simulink model "Robot_model_P_Control_ZOH_2025b"  (R2026a)
settings: Solver=VariableStepAuto  StopTime=10
values from neighbouring files (symbols this model uses):
  B = D * L    (= 9.682e-08)    [measurements.m]    (also in run_simulink.m = 0.15; run_simulink_PI_Controller.m = 0.15; run_simulink_turnrate_Controller.m = 0.15; run_simulink_turnrate_Controller_Heading.m = 0.15)
  D = 0.0000188    (= 1.88e-05)    [measurements.m]    (also in motor_model_m.m = 5e-05; run_simulink.m = 5e-05; run_simulink_PI_Controller.m = 5e-05; run_simulink_turnrate_Controller.m = 5e-05)
  J = -b / a    (= 2.25042607204e-06)    [measurements.m]    (also in motor_model_m.m = 5.56231644013e-06; run_simulink.m = 5.56231644013e-06; run_simulink_PI_Controller.m = 5.56231644013e-06; run_simulink_turnrate_Controller.m = 5.56231644013e-06)
  Kb = Kt    (= 0.009)    [motor_model_m.m]    (also in run_simulink.m; run_simulink_PI_Controller.m; run_simulink_turnrate_Controller.m; run_simulink_turnrate_Controller_Heading.m)
  Kp = 0.1202    [motor_model_m.m]    (also in run_simulink.m; run_simulink_PI_Controller.m; run_simulink_turnrate_Controller.m; run_simulink_turnrate_Controller_Heading.m)
  Kt = 0.009    [motor_model_m.m]    (also in run_simulink.m; run_simulink_PI_Controller.m; run_simulink_turnrate_Controller.m; run_simulink_turnrate_Controller_Heading.m)
  L = 5.15e-3    (= 0.00515)    [measurements.m]    (also in motor_model_m.m = 0.0045; run_simulink.m = 0.0045; run_simulink_PI_Controller.m = 0.0045; run_simulink_turnrate_Controller.m = 0.0045)
  mesDelay = 10*1e-3    (= 0.01)    [run_simulink.m]    (also in run_simulink_PI_Controller.m; run_simulink_turnrate_Controller.m; run_simulink_turnrate_Controller_Heading.m)
  R = 4.29    [measurements.m]    (also in motor_model_m.m; run_simulink.m; run_simulink_PI_Controller.m; run_simulink_turnrate_Controller.m)
  r2m = wheelRadius/gear    (= 0.00309917355372)    [motor_model_m.m]    (also in run_simulink.m; run_simulink_PI_Controller.m; run_simulink_turnrate_Controller.m; run_simulink_turnrate_Controller_Heading.m)
  Ts = 0.01    [run_simulink.m]    (also in run_simulink_PI_Controller.m; run_simulink_turnrate_Controller.m; run_simulink_turnrate_Controller_Heading.m)
settings Model: Creator=chr  LastModifiedBy=luma

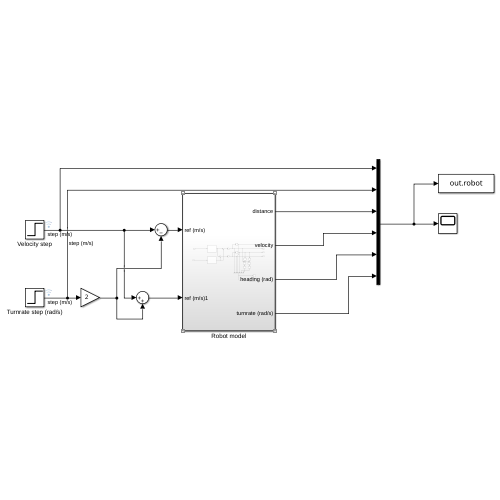
[thumbnail: Simulink's stored preview of the top-level diagram]
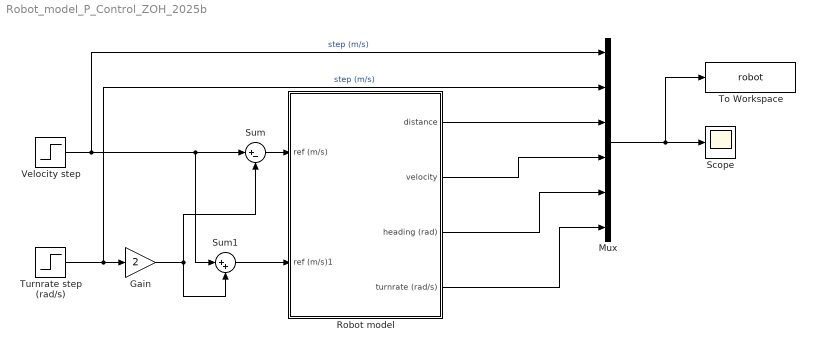
== system Robot_model_P_Control_ZOH_2025b ==
  Gain : Gain  Gain=2
  Mux : Mux  Inputs=6
  Robot model : Subsystem
  Scope : Scope
      settings: ActiveDisplayYMinimum=-13.33531780114458  ActiveDisplayYMaximum=120.01783697581038  DataLoggingVariableName=ScopeData2
  Sum : Sum  Inputs=|+-
  Sum1 : Sum  Inputs=|++
  To Workspace : ToWorkspace  VariableName=robot  SampleTime=-1
  Turnrate step (rad/s) : Step  Time=0.5  SampleTime=0
  Velocity step : Step  Time=0.1  FinalValue=0.6  SampleTime=0
  wires:
  Turnrate step (rad/s)/1 -> Mux/2, Gain/1  "step (m/s)"
  Gain/1 -> Sum/2, Sum1/2
  Velocity step/1 -> Mux/1, Sum1/1, Sum/1  "step (m/s)"
  Sum/1 -> Robot model/1(ref (m/s))
  Sum1/1 -> Robot model/2(ref (m/s)1)
  Robot model/1(distance) -> Mux/3
  Robot model/2(velocity) -> Mux/4
  Robot model/3(heading (rad)) -> Mux/5
  Robot model/4(turnrate (rad/s)) -> Mux/6
  Mux/1 -> To Workspace/1, Scope/1

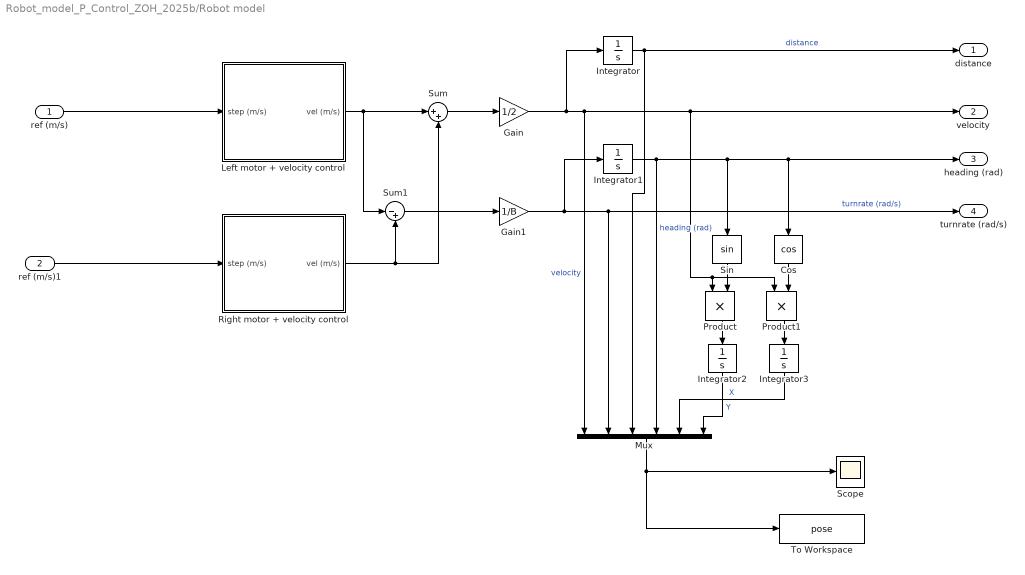
== system Robot_model_P_Control_ZOH_2025b/Robot model ==
  ref (m/s) : Inport
  ref (m/s)1 : Inport  Port=2
  Cos : Trigonometry  Operator=cos
  Gain : Gain  Gain=1/2
  Gain1 : Gain  Gain=1/B
  Integrator{,1..3} (4 alike) : Integrator
  "Left motor + velocity control " : Subsystem
  Mux : Mux  Inputs=6
  Product : Product
  Product1 : Product
  "Right motor + velocity control " : Subsystem
  Scope : Scope
      settings: ActiveDisplayYMinimum=-0.0093752663304982019  ActiveDisplayYMaximum=0.084377396974483834
  Sin : Trigonometry
  Sum : Sum  Inputs=|++
  Sum1 : Sum  Inputs=|-+
  To Workspace : ToWorkspace  VariableName=pose  SaveFormat=Timeseries  SampleTime=-1
  distance : Outport
  velocity : Outport  Port=2
  heading (rad) : Outport  Port=3
  turnrate (rad/s) : Outport  Port=4
  wires:
  Gain/1 -> Integrator/1, Mux/1, velocity/1, Product1/1, Product/1  "velocity"
  "Right motor + velocity control "/1(vel (m/s)) -> Sum/2, Sum1/2
  Mux/1 -> To Workspace/1, Scope/1
  Gain1/1 -> Integrator1/1, turnrate (rad/s)/1, Mux/2  "turnrate (rad/s)"
  Integrator3/1 -> Mux/5  "X"
  ref (m/s)1/1 -> "Right motor + velocity control "/1(step (m/s))
  Integrator/1 -> distance/1, Mux/3  "distance"
  "Left motor + velocity control "/1(vel (m/s)) -> Sum/1, Sum1/1
  ref (m/s)/1 -> "Left motor + velocity control "/1(step (m/s))
  Integrator1/1 -> Sin/1, heading (rad)/1, Cos/1, Mux/4  "heading (rad)"
  Sum1/1 -> Gain1/1
  Sum/1 -> Gain/1
  Product/1 -> Integrator2/1
  Cos/1 -> Product1/2
  Integrator2/1 -> Mux/6  "Y"
  Sin/1 -> Product/2
  Product1/1 -> Integrator3/1

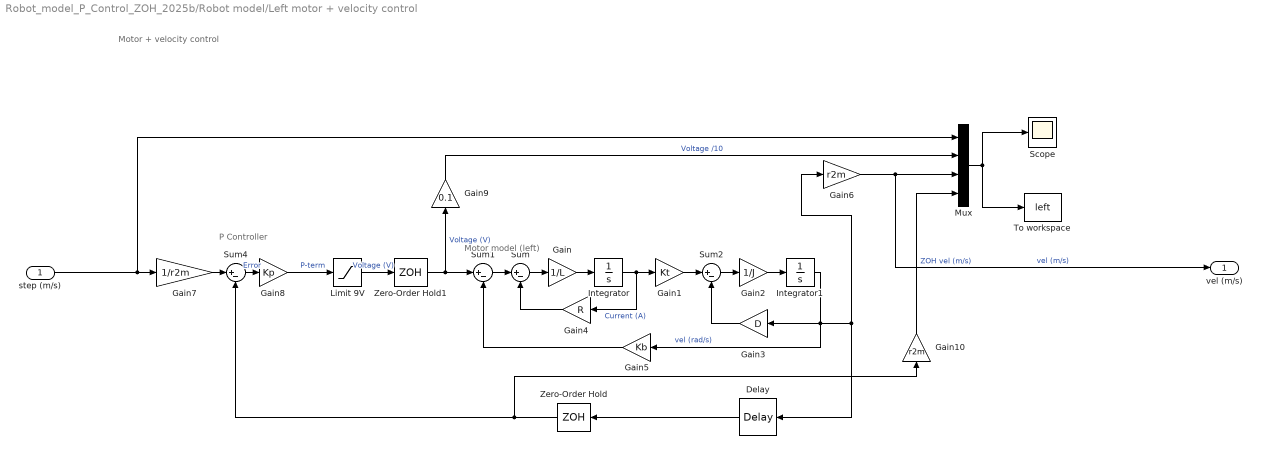
== system Robot_model_P_Control_ZOH_2025b/Robot model/Left motor + velocity control  ==
  note: Motor + velocity control
  note: P Controller
  note: Motor model (left)
  step (m/s) : Inport
  Delay : TransportDelay  DelayTime=mesDelay
  Gain : Gain  Gain=1/L
  Gain1 : Gain  Gain=Kt
  Gain10 : Gain  Gain=r2m
  Gain2 : Gain  Gain=1/J
  Gain3 : Gain  Gain=D
  Gain4 : Gain  Gain=R
  Gain5 : Gain  Gain=Kb
  Gain6 : Gain  Gain=r2m
  Gain7 : Gain  Gain=1/r2m
  Gain8 : Gain  Gain=Kp
  Gain9 : Gain  Gain=0.1
  Integrator : Integrator
  Integrator1 : Integrator
  Limit 9V : Saturate  UpperLimit=9  LowerLimit=-9
  Mux : Mux
  Scope : Scope
      settings: ActiveDisplayYMinimum=-0.28935  ActiveDisplayYMaximum=6.07084
  Sum{,1..2,4} (4 alike) : Sum  Inputs=|+-
  To workspace : ToWorkspace  VariableName=left  SaveFormat=Timeseries  SampleTime=-1
  Zero-Order Hold : ZeroOrderHold  SampleTime=Ts
  Zero-Order Hold1 : ZeroOrderHold  SampleTime=Ts
  vel (m/s) : Outport
  wires:
  Gain10/1 -> Mux/4  "ZOH vel (m/s)"
  Gain/1 -> Integrator/1
  Integrator1/1 -> Gain3/1, Gain5/1, Gain6/1, Delay/1  "vel (rad/s)"
  Gain7/1 -> Sum4/1
  Integrator/1 -> Gain4/1, Gain1/1  "Current (A)"
  step (m/s)/1 -> Mux/1, Gain7/1
  Gain5/1 -> Sum1/2
  Sum4/1 -> Gain8/1  "Error"
  Sum/1 -> Gain/1
  Gain2/1 -> Integrator1/1
  Gain8/1 -> Limit 9V/1  "P-term"
  Sum1/1 -> Sum/1
  Mux/1 -> Scope/1, To workspace/1
  Sum2/1 -> Gain2/1
  Gain3/1 -> Sum2/2
  Gain1/1 -> Sum2/1
  Gain6/1 -> vel (m/s)/1, Mux/3  "vel (m/s)"
  Zero-Order Hold/1 -> Gain10/1, Sum4/2
  Limit 9V/1 -> Zero-Order Hold1/1  "Voltage (V)"
  Zero-Order Hold1/1 -> Sum1/1, Gain9/1  "Voltage (V)"
  Delay/1 -> Zero-Order Hold/1
  Gain4/1 -> Sum/2
  Gain9/1 -> Mux/2  "Voltage /10"

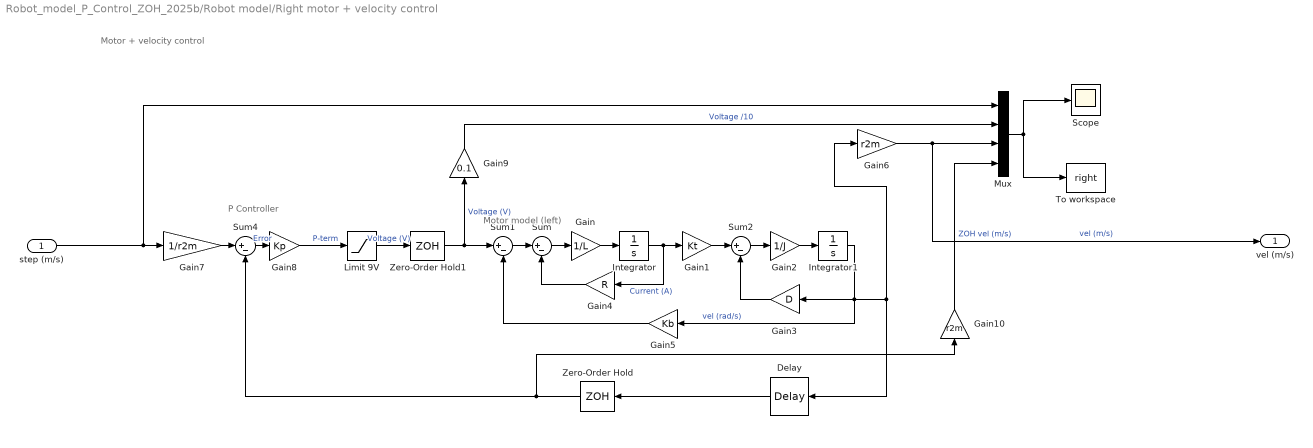
== system Robot_model_P_Control_ZOH_2025b/Robot model/Right motor + velocity control  ==
  note: Motor + velocity control
  note: Motor model (left)
  note: P Controller
  step (m/s) : Inport
  Delay : TransportDelay  DelayTime=mesDelay
  Gain : Gain  Gain=1/L
  Gain1 : Gain  Gain=Kt
  Gain10 : Gain  Gain=r2m
  Gain2 : Gain  Gain=1/J
  Gain3 : Gain  Gain=D
  Gain4 : Gain  Gain=R
  Gain5 : Gain  Gain=Kb
  Gain6 : Gain  Gain=r2m
  Gain7 : Gain  Gain=1/r2m
  Gain8 : Gain  Gain=Kp
  Gain9 : Gain  Gain=0.1
  Integrator : Integrator
  Integrator1 : Integrator
  Limit 9V : Saturate  UpperLimit=9  LowerLimit=-9
  Mux : Mux
  Scope : Scope
      settings: ActiveDisplayYMinimum=-0.28935  ActiveDisplayYMaximum=6.07084
  Sum{,1..2,4} (4 alike) : Sum  Inputs=|+-
  To workspace : ToWorkspace  VariableName=right  SaveFormat=Timeseries  SampleTime=-1
  Zero-Order Hold : ZeroOrderHold  SampleTime=Ts
  Zero-Order Hold1 : ZeroOrderHold  SampleTime=Ts
  vel (m/s) : Outport
  wires:
  Gain9/1 -> Mux/2  "Voltage /10"
  Gain4/1 -> Sum/2
  Delay/1 -> Zero-Order Hold/1
  Zero-Order Hold1/1 -> Gain9/1, Sum1/1  "Voltage (V)"
  Limit 9V/1 -> Zero-Order Hold1/1  "Voltage (V)"
  Zero-Order Hold/1 -> Sum4/2, Gain10/1
  Gain6/1 -> Mux/3, vel (m/s)/1  "vel (m/s)"
  Gain1/1 -> Sum2/1
  Gain3/1 -> Sum2/2
  Sum2/1 -> Gain2/1
  Mux/1 -> To workspace/1, Scope/1
  Sum1/1 -> Sum/1
  Gain8/1 -> Limit 9V/1  "P-term"
  Gain2/1 -> Integrator1/1
  Sum/1 -> Gain/1
  Sum4/1 -> Gain8/1  "Error"
  Gain5/1 -> Sum1/2
  step (m/s)/1 -> Gain7/1, Mux/1
  Integrator/1 -> Gain1/1, Gain4/1  "Current (A)"
  Gain7/1 -> Sum4/1
  Integrator1/1 -> Delay/1, Gain6/1, Gain5/1, Gain3/1  "vel (rad/s)"
  Gain/1 -> Integrator/1
  Gain10/1 -> Mux/4  "ZOH vel (m/s)"
